simulink model "sim_unicycle_model"  (R2025b)
settings: Solver=VariableStepAuto  StartTime=0.0  StopTime=10.0  RelTol=1e-3
libraries: simulink x1, robotmobilelib x1
settings Model: Creator=fatim  LastModifiedBy=fatim

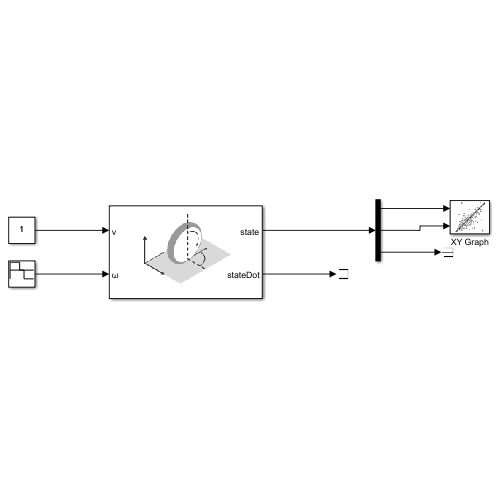
[thumbnail: Simulink's stored preview of the top-level diagram]
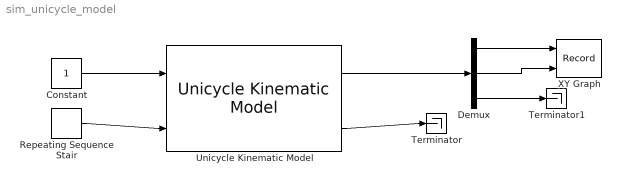
== system sim_unicycle_model ==
  Constant : Constant
  Demux : Demux  Outputs=3
  Repeating Sequence Stair : simulink/Sources/Repeating Sequence Stair  OutValues=[2 2 2 2 0 0 -2 -2 -2 -2]  tsamp=-1  OutMin=[]  OutMax=[]  OutDataTypeStr=double  OutputDataTypeScalingMode=double  OutDataType=fixdt(0,8)  ConRadixGroup=Best Precision: Vector-wise  OutScaling=2^-12
  Terminator : Terminator
  Terminator1 : Terminator
  Unicycle Kinematic Model : robotmobilelib/Unicycle Kinematic Model  VehicleInputs=Vehicle Speed & Heading Angular Velocity  WheelRadius=0.1  WheelSpeedRange=[-Inf Inf]  InitialState=[0; 0; 0]  SimulateUsing=Interpreted execution
  XY Graph : Record  NumPorts=2.0  FileSettingsInternal="{\"entries\":[{\"content\":{\"excelSettings\":{\"content\":{},\"type\":\"Streamout.ExcelSettings\"},\"parquetSettings\":{\"content\":{},\"type\":\"Streamout.ParquetSettings\"}},\"type\":\"Streamout.FileSettingStorage\",\"uuid\":\"\"}],\"packageUris\":[\"http:\\/\\/schema.mathworks.com\\/mf0\\/streamout_blocks\\/R2020a\"],\"version\":\"1.0\"}"  FrameSettings=[0, 0]  Layout=[1 1]  SignalsInternal="{\"entries\":[{\"content\":{\"signals\":[{\"content\":{\"blockPath\":[],\"dimensions\":[1],\"domain\":\"\",\"lineColor\":\"#a2142f\",\"plots\":[ 1 ],\"port\":1,\"sid\":[\"\"],\"signalID\":1,\"signalName\":\"Demux:1\"},\"type\":\"RecordBlkView.Signal\",\"uuid\":\"\"},{\"content\":{\"blockPath\":[],\"dimensions\":[1],\"domain\":\"\",\"lineColor\":\"#139fff\",\"plots\":[ 1 ],\"port\":2,\"sid\":[\"\"],\"signalID\":2,\"signalName\":\"Demux:2\"},\"type\":\"RecordBlkView.Signal\",\"uuid\":\"\"}]},\"type\":\"RecordBlkView.InputSignals\",\"uuid\":\"\"}],\"packageUris\":[\"http:\\/\\/schema.mathworks.com\\/mf0\\/streamout_blocks\\/R2020a\"],\"version\":\"1.0\"}"  VisualizationBindings="{\"xyplotplugin\":{\"info\":[{\"series\":[{\"bindingParametersList\":[{\"parameter\":\"X-Axis\",\"signalID\":1,\"signalName\":\"Demux:1\"},{\"parameter\":\"Y-Axis\",\"signalID\":2,\"signalName\":\"Demux:2\"}],\"seriesID\":0}],\"subplotID\":1}]}}"  CompatibilityTag=XY
  wires:
  Constant/1 -> Unicycle Kinematic Model/1
  Unicycle Kinematic Model/2 -> Terminator/1
  Unicycle Kinematic Model/1 -> Demux/1
  Demux/1 -> XY Graph/1
  Demux/2 -> XY Graph/2
  Demux/3 -> Terminator1/1
  Repeating Sequence Stair/1 -> Unicycle Kinematic Model/2
